simulink model "EV_Truck_Model"  (R2022b)
settings: Solver=FixedStepAuto  StartTime=0  StopTime=26553  FixedStep=0.1  RelTol=1e-3
model workspace (MAT data in the model file):
  ADAS_MaxAccel = 2
  ADAS_MaxDecel = 2.5
  Adas_on_off = 0
  Batt_cap_ah : Simulink.Parameter (value not decoded)
  Batt_rist_r0 : Simulink.Parameter (value not decoded)
  Batt_soc_s0 : Simulink.Parameter (value not decoded)
  Batt_volt_v0 : Simulink.Parameter (value not decoded)
  Motor_eff_100 : Simulink.Parameter (value not decoded)
  Motor_eff_190 : Simulink.Parameter (value not decoded)
  Motor_eff_95 : Simulink.Parameter (value not decoded)
  Motor_rpm_100 : Simulink.Parameter (value not decoded)
  Motor_rpm_190 : Simulink.Parameter (value not decoded)
  Motor_rpm_95 : Simulink.Parameter (value not decoded)
  Motor_torque_pos_100 : Simulink.Parameter (value not decoded)
  Motor_torque_pos_190 : Simulink.Parameter (value not decoded)
  Motor_torque_pos_95 : Simulink.Parameter (value not decoded)
  Motor_trq_190 : Simulink.Parameter (value not decoded)
  Motor_trq_95 : Simulink.Parameter (value not decoded)
  Sim_step = 0.1
  Test_DriveCycle = 0
  Trans_ratio = 6.142
  Veh_cog_fx = 1.69543
  Veh_cog_h = 0.605887
  Veh_cog_rx = 2.11956
  Veh_diff = 6.7
  Veh_whl_crr = 0.01
  Veh_whl_k = 180000
  Veh_whl_radius = 0.35
symbols that are objects in the model workspace (value not decoded): Motor_eff_100, Motor_eff_190, Motor_eff_95, Motor_rpm_100, Motor_rpm_190, Motor_rpm_95, Motor_torque_pos_100, Motor_torque_pos_190, Motor_torque_pos_95, Motor_trq_190, Motor_trq_95
undefined symbols (not defined in the file): Batt_soc_init, canChannel, Elec_aux_sw, Elec_rgn_sw, Power_option, speed, time, Veh_mass
libraries: batteryecm_lib x170, simulink x14, canmsglib x9, canlib x7, autolibshared x5, nesl_utility x4, fl_lib x3, drivingvehiclecontroller x3, hdlsllib x3, sim3dlib x1, sim3dautolib x1, vrlib x1
(part 10 of 11)

== system EV_Truck_Model/Accumulator System/Battery Pack/Simscape HV Battery/Battery Semi-Pack 4/Battery 7s6p5 ==
  Battery{1..7} (7 alike) : batteryecm_lib/Battery (Table-Based)  SOC_vec=Batt_soc_s0  T_dependence=simscape.enum.tablebattery.temperature_dependence.no  prm_dir=simscape.enum.tablebattery.prm_dir.noCurrentDirectionality  T_vec=[293] K  V0_mat=[2, 3, 3.2, 3.25, 3.25, 3.3, 3.3, 3.3, 3.35, 3.5] V  V0_vec=Batt_volt_v0 V  V_range=[0, inf] V  R0_mat=[15] mOhm  R0_vec=Batt_rist_r0 mOhm  R0_dis_mat=[.0117, .0085, .009; .011, .0085, .009; .0114, .0087, .0092; .0107, .0082, .0088; .0107, .0083, .0091; .0113, .0085, .0089; .0116, .0085, .0089] Ohm  R0_dis_vec=[.0085, .0085, .0087, .0082, .0083, .0085, .0085] Ohm  R0_ch_mat=[.0117, .0085, .009; .011, .0085, .009; .0114, .0087, .0092; .0107, .0082, .0088; .0107, .0083, .0091; .0113, .0085, .0089; .0116, .0085, .0089] Ohm  R0_ch_vec=[.0085, .0085, .0087, .0082, .0083, .0085, .0085] Ohm  AH=Batt_cap_ah A*hr  prm_leak=simscape.enum.tablebattery.prm_leak.disabled  Rleak_vec=[8000, 7000, 6000] Ohm  Rleak=7e3 Ohm  extrapolation_option=simscape.enum.extrapolation.nearest  SOC_port=simscape.enum.tablebattery.enable.no  prm_dyn=simscape.enum.tablebattery.prm_dyn.off  R1_mat=[.0109, .0029, .0013; .0069, .0024, .0012; .0047, .0026, .0013; .0034, .0016, .001; .0033, .0023, .0014; .0033, .0018, .0011; .0028, .0017, .0011] Ohm  R1_vec=[.0029, .0024, .0026, .0016, .0023, .0018, .0017] Ohm  tau1_mat=[20, 36, 39; 31, 45, 39; 109, 105, 61; 36, 29, 26; 59, 77, 67; 40, 33, 29; 25, 39, 33] s  tau1_vec=[36, 45, 105, 29, 77, 33, 39] s  R2_mat=[.0109, .0029, .0013; .0069, .0024, .0012; .0047, .0026, .0013; .0034, .0016, .001; .0033, .0023, .0014; .0033, .0018, .0011; .0028, .0017, .0011] Ohm  R2_vec=[.0029, .0024, .0026, .0016, .0023, .0018, .0017] Ohm  tau2_mat=[20, 36, 39; 31, 45, 39; 109, 105, 61; 36, 29, 26; 59, 77, 67; 40, 33, 29; 25, 39, 33] s  tau2_vec=[36, 45, 105, 29, 77, 33, 39] s  R3_mat=[.0109, .0029, .0013; .0069, .0024, .0012; .0047, .0026, .0013; .0034, .0016, .001; .0033, .0023, .0014; .0033, .0018, .0011; .0028, .0017, .0011] Ohm  R3_vec=[.0029, .0024, .0026, .0016, .0023, .0018, .0017] Ohm  tau3_mat=[20, 36, 39; 31, 45, 39; 109, 105, 61; 36, 29, 26; 59, 77, 67; 40, 33, 29; 25, 39, 33] s  tau3_vec=[36, 45, 105, 29, 77, 33, 39] s  R4_mat=[.0109, .0029, .0013; .0069, .0024, .0012; .0047, .0026, .0013; .0034, .0016, .001; .0033, .0023, .0014; .0033, .0018, .0011; .0028, .0017, .0011] Ohm  R4_vec=[.0029, .0024, .0026, .0016, .0023, .0018, .0017] Ohm  tau4_mat=[20, 36, 39; 31, 45, 39; 109, 105, 61; 36, 29, 26; 59, 77, 67; 40, 33, 29; 25, 39, 33] s  tau4_vec=[36, 45, 105, 29, 77, 33, 39] s  R5_mat=[.0109, .0029, .0013; .0069, .0024, .0012; .0047, .0026, .0013; .0034, .0016, .001; .0033, .0023, .0014; .0033, .0018, .0011; .0028, .0017, .0011] Ohm  R5_vec=[.0029, .0024, .0026, .0016, .0023, .0018, .0017] Ohm  tau5_mat=[20, 36, 39; 31, 45, 39; 109, 105, 61; 36, 29, 26; 59, 77, 67; 40, 33, 29; 25, 39, 33] s  tau5_vec=[36, 45, 105, 29, 77, 33, 39] s  prm_fade=simscape.enum.tablebattery.prm_fade.disabled  N0=100  dV0=0  dR0=0  dAH=0  dRleak=0  dR1=0  dR2=0  dR3=0  dR4=0  dR5=0  N0vec=[100, 200, 300]  Tfadevec=[298.15, 323.15] K  dV0vec=[0, 0, 0]  dR0vec=[0, 0, 0]  dAHvec=[0, 0, 0]  dRleakvec=[0, 0, 0]  dR1vec=[0, 0, 0]  dR2vec=[0, 0, 0]  dR3vec=[0, 0, 0]  dR4vec=[0, 0, 0]  dR5vec=[0, 0, 0]  dV0mat=[0, 0; 0, 0; 0, 0]  dR0mat=[0, 0; 0, 0; 0, 0]  dAHmat=[0, 0; 0, 0; 0, 0]  dRleakmat=[0, 0; 0, 0; 0, 0]  dR1mat=[0, 0; 0, 0; 0, 0]  dR2mat=[0, 0; 0, 0; 0, 0]  dR3mat=[0, 0; 0, 0; 0, 0]  dR4mat=[0, 0; 0, 0; 0, 0]  dR5mat=[0, 0; 0, 0; 0, 0]  prm_age_modeling=simscape.enum.tablebattery.prm_age_modeling.equation  storage_dt_age_vec=[0] d  storage_T_age_vec=[273] K  prm_age_OCV=simscape.enum.tablebattery.prm_age_OCV.OCV  OCV_age=0.9  SOC_age=0.6  prm_age_resistance=simscape.enum.tablebattery.prm_age.disabled  OCV_scaling_age_resistance=2.2134e6  OCV_offset_age_resistance=1.632e6  temp_exp_age_resistance=0.515833569 V  t_exp_age_resistance=0.75  T_age_vec_resistance=[273.15, 298.15, 323.15] K  dt_age_vec_resistance=[90, 180, 270, 360] d  dR0_age_vec=[0, 0, 0]  t_meas_dR0_age=100 d  dR0_age_mat=[0, 0, 0; 0, 0, 0; 0, 0, 0; 0, 0, 0]  prm_age_capacity=simscape.enum.tablebattery.prm_age.disabled  OCV_scaling_age_capacity=1.5097e07  OCV_offset_age_capacity=8.3625e06  temp_exp_age_capacity=0.6011 V  t_exp_age_capacity=0.75  T_age_vec_capacity=[273.15, 298.15, 323.15] K  dt_age_vec_capacity=[90, 180, 270, 360] d  dAH_age_vec=[0, 0, 0]  t_meas_dAH_age=100 d  dAH_age_mat=[0, 0, 0; 0, 0, 0; 0, 0, 0; 0, 0, 0]  thermal_port=simscape.enum.thermaleffects.omit  temperature=298.15 K  thermal_mass=100 J/K  i_specify=off  i_priority=None  i=0 A  i_nominal_specify=off  i_nominal_unit=A  i_nominal_value=1  v_specify=off  v_priority=None  v=0 V  v_nominal_specify=off  v_nominal_unit=V  v_nominal_value=1  stateOfCharge_specify=on  stateOfCharge_priority=High  stateOfCharge=Batt_soc_init  stateOfCharge_nominal_specify=off  stateOfCharge_nominal_unit=1  stateOfCharge_nominal_value=1  num_cycles_specify=off  num_cycles_priority=High  num_cycles=0  num_cycles_nominal_specify=off  num_cycles_nominal_unit=1  num_cycles_nominal_value=1  cell_temperature_specify=off  cell_temperature_priority=High  cell_temperature=298.15 K  cell_temperature_nominal_specify=off  cell_temperature_nominal_unit=K  cell_temperature_nominal_value=1
      settings: InternalSimscapePortConfiguration="{\"Bottom\":[],\"Left\":[{\"id\":\"p\",\"label\":\"+\",\"type\":\"foundation.electrical.electrical\"}],\"Right\":[{\"id\":\"n\",\"label\":\"-\",\"type\":\"foundation.electrical.electrical\"}],\"Top\":[]}"
  High : PMIOPort  Side=Left
  Low : PMIOPort  Port=2  Side=Right
  connections:
  Low/RConn1 -- Battery7/RConn1
  Battery1/LConn1 -- High/RConn1
  Battery2/LConn1 -- Battery1/RConn1
  Battery3/LConn1 -- Battery2/RConn1
  Battery4/LConn1 -- Battery3/RConn1
  Battery5/LConn1 -- Battery4/RConn1
  Battery6/LConn1 -- Battery5/RConn1
  Battery7/LConn1 -- Battery6/RConn1

== system EV_Truck_Model/Accumulator System/Battery Pack/Simscape HV Battery/Battery Semi-Pack 4/Battery 7s6p6 ==
  Battery{1..6} (6 alike) : batteryecm_lib/Battery (Table-Based)  SOC_vec=Batt_soc_s0  T_dependence=simscape.enum.tablebattery.temperature_dependence.no  prm_dir=simscape.enum.tablebattery.prm_dir.noCurrentDirectionality  T_vec=[293] K  V0_mat=[2, 3, 3.2, 3.25, 3.25, 3.3, 3.3, 3.3, 3.35, 3.5] V  V0_vec=Batt_volt_v0 V  V_range=[0, inf] V  R0_mat=[15] mOhm  R0_vec=Batt_rist_r0 mOhm  R0_dis_mat=[.0117, .0085, .009; .011, .0085, .009; .0114, .0087, .0092; .0107, .0082, .0088; .0107, .0083, .0091; .0113, .0085, .0089; .0116, .0085, .0089] Ohm  R0_dis_vec=[.0085, .0085, .0087, .0082, .0083, .0085, .0085] Ohm  R0_ch_mat=[.0117, .0085, .009; .011, .0085, .009; .0114, .0087, .0092; .0107, .0082, .0088; .0107, .0083, .0091; .0113, .0085, .0089; .0116, .0085, .0089] Ohm  R0_ch_vec=[.0085, .0085, .0087, .0082, .0083, .0085, .0085] Ohm  AH=Batt_cap_ah A*hr  prm_leak=simscape.enum.tablebattery.prm_leak.disabled  Rleak_vec=[8000, 7000, 6000] Ohm  Rleak=7e3 Ohm  extrapolation_option=simscape.enum.extrapolation.nearest  SOC_port=simscape.enum.tablebattery.enable.no  prm_dyn=simscape.enum.tablebattery.prm_dyn.off  R1_mat=[.0109, .0029, .0013; .0069, .0024, .0012; .0047, .0026, .0013; .0034, .0016, .001; .0033, .0023, .0014; .0033, .0018, .0011; .0028, .0017, .0011] Ohm  R1_vec=[.0029, .0024, .0026, .0016, .0023, .0018, .0017] Ohm  tau1_mat=[20, 36, 39; 31, 45, 39; 109, 105, 61; 36, 29, 26; 59, 77, 67; 40, 33, 29; 25, 39, 33] s  tau1_vec=[36, 45, 105, 29, 77, 33, 39] s  R2_mat=[.0109, .0029, .0013; .0069, .0024, .0012; .0047, .0026, .0013; .0034, .0016, .001; .0033, .0023, .0014; .0033, .0018, .0011; .0028, .0017, .0011] Ohm  R2_vec=[.0029, .0024, .0026, .0016, .0023, .0018, .0017] Ohm  tau2_mat=[20, 36, 39; 31, 45, 39; 109, 105, 61; 36, 29, 26; 59, 77, 67; 40, 33, 29; 25, 39, 33] s  tau2_vec=[36, 45, 105, 29, 77, 33, 39] s  R3_mat=[.0109, .0029, .0013; .0069, .0024, .0012; .0047, .0026, .0013; .0034, .0016, .001; .0033, .0023, .0014; .0033, .0018, .0011; .0028, .0017, .0011] Ohm  R3_vec=[.0029, .0024, .0026, .0016, .0023, .0018, .0017] Ohm  tau3_mat=[20, 36, 39; 31, 45, 39; 109, 105, 61; 36, 29, 26; 59, 77, 67; 40, 33, 29; 25, 39, 33] s  tau3_vec=[36, 45, 105, 29, 77, 33, 39] s  R4_mat=[.0109, .0029, .0013; .0069, .0024, .0012; .0047, .0026, .0013; .0034, .0016, .001; .0033, .0023, .0014; .0033, .0018, .0011; .0028, .0017, .0011] Ohm  R4_vec=[.0029, .0024, .0026, .0016, .0023, .0018, .0017] Ohm  tau4_mat=[20, 36, 39; 31, 45, 39; 109, 105, 61; 36, 29, 26; 59, 77, 67; 40, 33, 29; 25, 39, 33] s  tau4_vec=[36, 45, 105, 29, 77, 33, 39] s  R5_mat=[.0109, .0029, .0013; .0069, .0024, .0012; .0047, .0026, .0013; .0034, .0016, .001; .0033, .0023, .0014; .0033, .0018, .0011; .0028, .0017, .0011] Ohm  R5_vec=[.0029, .0024, .0026, .0016, .0023, .0018, .0017] Ohm  tau5_mat=[20, 36, 39; 31, 45, 39; 109, 105, 61; 36, 29, 26; 59, 77, 67; 40, 33, 29; 25, 39, 33] s  tau5_vec=[36, 45, 105, 29, 77, 33, 39] s  prm_fade=simscape.enum.tablebattery.prm_fade.disabled  N0=100  dV0=0  dR0=0  dAH=0  dRleak=0  dR1=0  dR2=0  dR3=0  dR4=0  dR5=0  N0vec=[100, 200, 300]  Tfadevec=[298.15, 323.15] K  dV0vec=[0, 0, 0]  dR0vec=[0, 0, 0]  dAHvec=[0, 0, 0]  dRleakvec=[0, 0, 0]  dR1vec=[0, 0, 0]  dR2vec=[0, 0, 0]  dR3vec=[0, 0, 0]  dR4vec=[0, 0, 0]  dR5vec=[0, 0, 0]  dV0mat=[0, 0; 0, 0; 0, 0]  dR0mat=[0, 0; 0, 0; 0, 0]  dAHmat=[0, 0; 0, 0; 0, 0]  dRleakmat=[0, 0; 0, 0; 0, 0]  dR1mat=[0, 0; 0, 0; 0, 0]  dR2mat=[0, 0; 0, 0; 0, 0]  dR3mat=[0, 0; 0, 0; 0, 0]  dR4mat=[0, 0; 0, 0; 0, 0]  dR5mat=[0, 0; 0, 0; 0, 0]  prm_age_modeling=simscape.enum.tablebattery.prm_age_modeling.equation  storage_dt_age_vec=[0] d  storage_T_age_vec=[273] K  prm_age_OCV=simscape.enum.tablebattery.prm_age_OCV.OCV  OCV_age=0.9  SOC_age=0.6  prm_age_resistance=simscape.enum.tablebattery.prm_age.disabled  OCV_scaling_age_resistance=2.2134e6  OCV_offset_age_resistance=1.632e6  temp_exp_age_resistance=0.515833569 V  t_exp_age_resistance=0.75  T_age_vec_resistance=[273.15, 298.15, 323.15] K  dt_age_vec_resistance=[90, 180, 270, 360] d  dR0_age_vec=[0, 0, 0]  t_meas_dR0_age=100 d  dR0_age_mat=[0, 0, 0; 0, 0, 0; 0, 0, 0; 0, 0, 0]  prm_age_capacity=simscape.enum.tablebattery.prm_age.disabled  OCV_scaling_age_capacity=1.5097e07  OCV_offset_age_capacity=8.3625e06  temp_exp_age_capacity=0.6011 V  t_exp_age_capacity=0.75  T_age_vec_capacity=[273.15, 298.15, 323.15] K  dt_age_vec_capacity=[90, 180, 270, 360] d  dAH_age_vec=[0, 0, 0]  t_meas_dAH_age=100 d  dAH_age_mat=[0, 0, 0; 0, 0, 0; 0, 0, 0; 0, 0, 0]  thermal_port=simscape.enum.thermaleffects.omit  temperature=298.15 K  thermal_mass=100 J/K  i_specify=off  i_priority=None  i=0 A  i_nominal_specify=off  i_nominal_unit=A  i_nominal_value=1  v_specify=off  v_priority=None  v=0 V  v_nominal_specify=off  v_nominal_unit=V  v_nominal_value=1  stateOfCharge_specify=on  stateOfCharge_priority=High  stateOfCharge=Batt_soc_init  stateOfCharge_nominal_specify=off  stateOfCharge_nominal_unit=1  stateOfCharge_nominal_value=1  num_cycles_specify=off  num_cycles_priority=High  num_cycles=0  num_cycles_nominal_specify=off  num_cycles_nominal_unit=1  num_cycles_nominal_value=1  cell_temperature_specify=off  cell_temperature_priority=High  cell_temperature=298.15 K  cell_temperature_nominal_specify=off  cell_temperature_nominal_unit=K  cell_temperature_nominal_value=1
      settings: InternalSimscapePortConfiguration="{\"Bottom\":[],\"Left\":[{\"id\":\"p\",\"label\":\"+\",\"type\":\"foundation.electrical.electrical\"}],\"Right\":[{\"id\":\"n\",\"label\":\"-\",\"type\":\"foundation.electrical.electrical\"}],\"Top\":[]}"
  Battery7 : batteryecm_lib/Battery (Table-Based)  SOC_vec=Batt_soc_s0  T_dependence=simscape.enum.tablebattery.temperature_dependence.no  prm_dir=simscape.enum.tablebattery.prm_dir.noCurrentDirectionality  T_vec=[293] K  V0_mat=[2, 3, 3.2, 3.25, 3.25, 3.3, 3.3, 3.3, 3.35, 3.5] V  V0_vec=Batt_volt_v0 V  V_range=[0, inf] V  R0_mat=[15] mOhm  R0_vec=Batt_rist_r0 mOhm  R0_dis_mat=[.0117, .0085, .009; .011, .0085, .009; .0114, .0087, .0092; .0107, .0082, .0088; .0107, .0083, .0091; .0113, .0085, .0089; .0116, .0085, .0089] Ohm  R0_dis_vec=[.0085, .0085, .0087, .0082, .0083, .0085, .0085] Ohm  R0_ch_mat=[.0117, .0085, .009; .011, .0085, .009; .0114, .0087, .0092; .0107, .0082, .0088; .0107, .0083, .0091; .0113, .0085, .0089; .0116, .0085, .0089] Ohm  R0_ch_vec=[.0085, .0085, .0087, .0082, .0083, .0085, .0085] Ohm  AH=Batt_cap_ah A*hr  prm_leak=simscape.enum.tablebattery.prm_leak.disabled  Rleak_vec=[8000, 7000, 6000] Ohm  Rleak=7e3 Ohm  extrapolation_option=simscape.enum.extrapolation.nearest  SOC_port=simscape.enum.tablebattery.enable.yes  prm_dyn=simscape.enum.tablebattery.prm_dyn.off  R1_mat=[.0109, .0029, .0013; .0069, .0024, .0012; .0047, .0026, .0013; .0034, .0016, .001; .0033, .0023, .0014; .0033, .0018, .0011; .0028, .0017, .0011] Ohm  R1_vec=[.0029, .0024, .0026, .0016, .0023, .0018, .0017] Ohm  tau1_mat=[20, 36, 39; 31, 45, 39; 109, 105, 61; 36, 29, 26; 59, 77, 67; 40, 33, 29; 25, 39, 33] s  tau1_vec=[36, 45, 105, 29, 77, 33, 39] s  R2_mat=[.0109, .0029, .0013; .0069, .0024, .0012; .0047, .0026, .0013; .0034, .0016, .001; .0033, .0023, .0014; .0033, .0018, .0011; .0028, .0017, .0011] Ohm  R2_vec=[.0029, .0024, .0026, .0016, .0023, .0018, .0017] Ohm  tau2_mat=[20, 36, 39; 31, 45, 39; 109, 105, 61; 36, 29, 26; 59, 77, 67; 40, 33, 29; 25, 39, 33] s  tau2_vec=[36, 45, 105, 29, 77, 33, 39] s  R3_mat=[.0109, .0029, .0013; .0069, .0024, .0012; .0047, .0026, .0013; .0034, .0016, .001; .0033, .0023, .0014; .0033, .0018, .0011; .0028, .0017, .0011] Ohm  R3_vec=[.0029, .0024, .0026, .0016, .0023, .0018, .0017] Ohm  tau3_mat=[20, 36, 39; 31, 45, 39; 109, 105, 61; 36, 29, 26; 59, 77, 67; 40, 33, 29; 25, 39, 33] s  tau3_vec=[36, 45, 105, 29, 77, 33, 39] s  R4_mat=[.0109, .0029, .0013; .0069, .0024, .0012; .0047, .0026, .0013; .0034, .0016, .001; .0033, .0023, .0014; .0033, .0018, .0011; .0028, .0017, .0011] Ohm  R4_vec=[.0029, .0024, .0026, .0016, .0023, .0018, .0017] Ohm  tau4_mat=[20, 36, 39; 31, 45, 39; 109, 105, 61; 36, 29, 26; 59, 77, 67; 40, 33, 29; 25, 39, 33] s  tau4_vec=[36, 45, 105, 29, 77, 33, 39] s  R5_mat=[.0109, .0029, .0013; .0069, .0024, .0012; .0047, .0026, .0013; .0034, .0016, .001; .0033, .0023, .0014; .0033, .0018, .0011; .0028, .0017, .0011] Ohm  R5_vec=[.0029, .0024, .0026, .0016, .0023, .0018, .0017] Ohm  tau5_mat=[20, 36, 39; 31, 45, 39; 109, 105, 61; 36, 29, 26; 59, 77, 67; 40, 33, 29; 25, 39, 33] s  tau5_vec=[36, 45, 105, 29, 77, 33, 39] s  prm_fade=simscape.enum.tablebattery.prm_fade.disabled  N0=100  dV0=0  dR0=0  dAH=0  dRleak=0  dR1=0  dR2=0  dR3=0  dR4=0  dR5=0  N0vec=[100, 200, 300]  Tfadevec=[298.15, 323.15] K  dV0vec=[0, 0, 0]  dR0vec=[0, 0, 0]  dAHvec=[0, 0, 0]  dRleakvec=[0, 0, 0]  dR1vec=[0, 0, 0]  dR2vec=[0, 0, 0]  dR3vec=[0, 0, 0]  dR4vec=[0, 0, 0]  dR5vec=[0, 0, 0]  dV0mat=[0, 0; 0, 0; 0, 0]  dR0mat=[0, 0; 0, 0; 0, 0]  dAHmat=[0, 0; 0, 0; 0, 0]  dRleakmat=[0, 0; 0, 0; 0, 0]  dR1mat=[0, 0; 0, 0; 0, 0]  dR2mat=[0, 0; 0, 0; 0, 0]  dR3mat=[0, 0; 0, 0; 0, 0]  dR4mat=[0, 0; 0, 0; 0, 0]  dR5mat=[0, 0; 0, 0; 0, 0]  prm_age_modeling=simscape.enum.tablebattery.prm_age_modeling.equation  storage_dt_age_vec=[0] d  storage_T_age_vec=[273] K  prm_age_OCV=simscape.enum.tablebattery.prm_age_OCV.OCV  OCV_age=0.9  SOC_age=0.6  prm_age_resistance=simscape.enum.tablebattery.prm_age.disabled  OCV_scaling_age_resistance=2.2134e6  OCV_offset_age_resistance=1.632e6  temp_exp_age_resistance=0.515833569 V  t_exp_age_resistance=0.75  T_age_vec_resistance=[273.15, 298.15, 323.15] K  dt_age_vec_resistance=[90, 180, 270, 360] d  dR0_age_vec=[0, 0, 0]  t_meas_dR0_age=100 d  dR0_age_mat=[0, 0, 0; 0, 0, 0; 0, 0, 0; 0, 0, 0]  prm_age_capacity=simscape.enum.tablebattery.prm_age.disabled  OCV_scaling_age_capacity=1.5097e07  OCV_offset_age_capacity=8.3625e06  temp_exp_age_capacity=0.6011 V  t_exp_age_capacity=0.75  T_age_vec_capacity=[273.15, 298.15, 323.15] K  dt_age_vec_capacity=[90, 180, 270, 360] d  dAH_age_vec=[0, 0, 0]  t_meas_dAH_age=100 d  dAH_age_mat=[0, 0, 0; 0, 0, 0; 0, 0, 0; 0, 0, 0]  thermal_port=simscape.enum.thermaleffects.omit  temperature=298.15 K  thermal_mass=100 J/K  i_specify=off  i_priority=None  i=0 A  i_nominal_specify=off  i_nominal_unit=A  i_nominal_value=1  v_specify=off  v_priority=None  v=0 V  v_nominal_specify=off  v_nominal_unit=V  v_nominal_value=1  stateOfCharge_specify=on  stateOfCharge_priority=High  stateOfCharge=Batt_soc_init  stateOfCharge_nominal_specify=off  stateOfCharge_nominal_unit=1  stateOfCharge_nominal_value=1  num_cycles_specify=off  num_cycles_priority=High  num_cycles=0  num_cycles_nominal_specify=off  num_cycles_nominal_unit=1  num_cycles_nominal_value=1  cell_temperature_specify=off  cell_temperature_priority=High  cell_temperature=298.15 K  cell_temperature_nominal_specify=off  cell_temperature_nominal_unit=K  cell_temperature_nominal_value=1
      settings: InternalSimscapePortConfiguration="{\"Bottom\":[],\"Left\":[{\"id\":\"p\",\"label\":\"+\",\"type\":\"foundation.electrical.electrical\"},{\"id\":\"soc\",\"label\":\"SOC\",\"type\":\"output\"}],\"Right\":[{\"id\":\"n\",\"label\":\"-\",\"type\":\"foundation.electrical.electrical\"}],\"Top\":[]}"
  High : PMIOPort  Side=Left
  Low : PMIOPort  Port=2  Side=Right
  SOC : PMIOPort  Port=3  Side=Left
  connections:
  Low/RConn1 -- Battery7/RConn1
  Battery1/LConn1 -- High/RConn1
  Battery2/LConn1 -- Battery1/RConn1
  Battery3/LConn1 -- Battery2/RConn1
  Battery4/LConn1 -- Battery3/RConn1
  Battery5/LConn1 -- Battery4/RConn1
  Battery6/LConn1 -- Battery5/RConn1
  Battery7/LConn1 -- Battery6/RConn1
  Battery7/LConn2 -- SOC/RConn1

== system EV_Truck_Model/VCU/Remap Subsystem/Longitudinal Control Subsystem/If Action Subsystem/ADAS Torque Command MUX ==
  TrqCmd : Inport
  BrakeCmd : Inport  Port=2
  TrqCmd_ADAS : Inport  Port=3
  BrakeCmd_ADAS : Inport  Port=4
  Constant : Constant  Value=0
  If : If  IfExpression=u1 == 1
  If Action Subsystem : Subsystem  TreatAsAtomicUnit=on
  If Action Subsystem1 : Subsystem  TreatAsAtomicUnit=on
  Merge : Merge
  Merge1 : Merge
  TrqCmd_MUX : Outport
  BrakeCmd_MUX : Outport  Port=2
  wires:
  TrqCmd/1 -> If Action Subsystem/1(TrqCmd)
  If Action Subsystem/1(Out1) -> Merge/1
  TrqCmd_ADAS/1 -> If Action Subsystem1/1(TrqCmd_ADAS)
  If Action Subsystem1/1(Out1) -> Merge/2
  Constant/1 -> If/1
  If/1 -> If Action Subsystem1/Action
  If/2 -> If Action Subsystem/Action
  Merge/1 -> TrqCmd_MUX/1
  BrakeCmd/1 -> If Action Subsystem/2(BrakeCmd)
  BrakeCmd_ADAS/1 -> If Action Subsystem1/2(BrakeCmd_ADAS)
  Merge1/1 -> BrakeCmd_MUX/1
  If Action Subsystem1/2(Out2) -> Merge1/2
  If Action Subsystem/2(Out2) -> Merge1/1

== system EV_Truck_Model/VCU/Remap Subsystem/Longitudinal Controller/ADAS Torque Command MUX/If Action Subsystem ==
  TrqCmd : Inport
  BrakeCmd : Inport  Port=2
  Action Port : ActionPort  ActionPortLabel=else
  Out1 : Outport
  Out2 : Outport  Port=2
  wires:
  TrqCmd/1 -> Out1/1
  BrakeCmd/1 -> Out2/1

== system EV_Truck_Model/VCU/Remap Subsystem/Longitudinal Controller/ADAS Torque Command MUX/If Action Subsystem1 ==
  TrqCmd_ADAS : Inport
  BrakeCmd_ADAS : Inport  Port=2
  Action Port : ActionPort  ActionPortLabel=if(u1 == 1)
  Out1 : Outport
  Out2 : Outport  Port=2
  wires:
  TrqCmd_ADAS/1 -> Out1/1
  BrakeCmd_ADAS/1 -> Out2/1

== system EV_Truck_Model/VCU/Remap Subsystem/TTC Calculator/Subsystem/Subsystem ==
  In1 : Inport
  In2 : Inport  Port=2
  Constant : Constant
  Delay : Delay  DelayLengthSource=Input port  DelayLength=1
      settings: InputPortMap=u0,p1
  Delay1 : Delay  DelayLengthSource=Input port  DelayLength=1
      settings: InputPortMap=u0,p1
  Divide : Product  Inputs=*/
  Minus : Sum  Inputs=+-
  Minus1 : Sum  Inputs=+-
  Out1 : Outport
  wires:
  Minus/1 -> Divide/1
  Delay/1 -> Minus/2
  In1/1 -> Minus/1, Delay/1
  Delay1/1 -> Minus1/2
  In2/1 -> Delay1/1, Minus1/1
  Minus1/1 -> Divide/2
  Divide/1 -> Out1/1
  Constant/1 -> Delay1/2, Delay/2

== system EV_Truck_Model/VCU/Remap Subsystem/TTC Calculator/Subsystem/Subsystem1 ==
  In1 : Inport
  In2 : Inport  Port=2
  Constant : Constant  Value=2
  Delay : Delay  DelayLengthSource=Input port  DelayLength=1
      settings: InputPortMap=u0,p1
  Delay1 : Delay  DelayLengthSource=Input port  DelayLength=1
      settings: InputPortMap=u0,p1
  Divide : Product  Inputs=*/
  Minus : Sum  Inputs=+-
  Minus1 : Sum  Inputs=+-
  Out1 : Outport
  wires:
  Minus/1 -> Divide/1
  Delay/1 -> Minus/2
  In1/1 -> Minus/1, Delay/1
  Delay1/1 -> Minus1/2
  In2/1 -> Delay1/1, Minus1/1
  Minus1/1 -> Divide/2
  Divide/1 -> Out1/1
  Constant/1 -> Delay1/2, Delay/2

== system EV_Truck_Model/VCU/Remap Subsystem/TTC Calculator/Subsystem/Subsystem2 ==
  In1 : Inport
  In2 : Inport  Port=2
  Constant : Constant  Value=3
  Delay : Delay  DelayLengthSource=Input port  DelayLength=1
      settings: InputPortMap=u0,p1
  Delay1 : Delay  DelayLengthSource=Input port  DelayLength=1
      settings: InputPortMap=u0,p1
  Divide : Product  Inputs=*/
  Minus : Sum  Inputs=+-
  Minus1 : Sum  Inputs=+-
  Out1 : Outport
  wires:
  Minus/1 -> Divide/1
  Delay/1 -> Minus/2
  In1/1 -> Minus/1, Delay/1
  Delay1/1 -> Minus1/2
  In2/1 -> Delay1/1, Minus1/1
  Minus1/1 -> Divide/2
  Divide/1 -> Out1/1
  Constant/1 -> Delay1/2, Delay/2

== system EV_Truck_Model/VCU/Remap Subsystem/TTC Calculator/Subsystem/Subsystem3 ==
  In1 : Inport
  In2 : Inport  Port=2
  Constant : Constant  Value=4
  Delay : Delay  DelayLengthSource=Input port  DelayLength=1
      settings: InputPortMap=u0,p1
  Delay1 : Delay  DelayLengthSource=Input port  DelayLength=1
      settings: InputPortMap=u0,p1
  Divide : Product  Inputs=*/
  Minus : Sum  Inputs=+-
  Minus1 : Sum  Inputs=+-
  Out1 : Outport
  wires:
  Minus/1 -> Divide/1
  Delay/1 -> Minus/2
  In1/1 -> Minus/1, Delay/1
  Delay1/1 -> Minus1/2
  In2/1 -> Delay1/1, Minus1/1
  Minus1/1 -> Divide/2
  Divide/1 -> Out1/1
  Constant/1 -> Delay1/2, Delay/2

== system EV_Truck_Model/VCU/Remap Subsystem/TTC Calculator/Subsystem/Subsystem4 ==
  In1 : Inport
  In2 : Inport  Port=2
  Constant : Constant  Value=5
  Delay : Delay  DelayLengthSource=Input port  DelayLength=1
      settings: InputPortMap=u0,p1
  Delay1 : Delay  DelayLengthSource=Input port  DelayLength=1
      settings: InputPortMap=u0,p1
  Divide : Product  Inputs=*/
  Minus : Sum  Inputs=+-
  Minus1 : Sum  Inputs=+-
  Out1 : Outport
  wires:
  Minus/1 -> Divide/1
  Delay/1 -> Minus/2
  In1/1 -> Minus/1, Delay/1
  Delay1/1 -> Minus1/2
  In2/1 -> Delay1/1, Minus1/1
  Minus1/1 -> Divide/2
  Divide/1 -> Out1/1
  Constant/1 -> Delay1/2, Delay/2

== system EV_Truck_Model/Vehicle Dynamics System/Power Delivery and Braking System/BrakeSystem & Tyre Rolling Resistance/Subsystem/If Action Subsystem ==
  MotorSpeed : Inport
  BrakingForce : Inport  Port=2
  Action Port : ActionPort  ActionPortLabel=if((-125 < u1) & (u1 < 125))
  Multiply : Gain  Gain=-1/125
  multiply : Product  Inputs=**
  Out1 : Outport
  wires:
  multiply/1 -> Multiply/1
  BrakingForce/1 -> multiply/2
  MotorSpeed/1 -> multiply/1
  Multiply/1 -> Out1/1

== system EV_Truck_Model/Vehicle Dynamics System/Power Delivery and Braking System/BrakeSystem & Tyre Rolling Resistance/Subsystem/If Action Subsystem1 ==
  BrakingForce : Inport
  Action Port : ActionPort  ActionPortLabel=elseif(u1 > 0)
  Multiply : Gain  Gain=-1
  Out1 : Outport
  wires:
  BrakingForce/1 -> Multiply/1
  Multiply/1 -> Out1/1

== system EV_Truck_Model/Vehicle Dynamics System/Power Delivery and Braking System/BrakeSystem & Tyre Rolling Resistance/Subsystem/If Action Subsystem2 ==
  BrakingForce : Inport
  Action Port : ActionPort  ActionPortLabel=elseif(u1 < 0)
  Multiply : Gain
  Out1 : Outport
  wires:
  BrakingForce/1 -> Multiply/1
  Multiply/1 -> Out1/1

== system EV_Truck_Model/VCU/Remap Subsystem/Longitudinal Control Subsystem/If Action Subsystem/ADAS Torque Command MUX/If Action Subsystem ==
  TrqCmd : Inport
  BrakeCmd : Inport  Port=2
  Action Port : ActionPort
  Out1 : Outport
  Out2 : Outport  Port=2
  wires:
  TrqCmd/1 -> Out1/1
  BrakeCmd/1 -> Out2/1

== system EV_Truck_Model/VCU/Remap Subsystem/Longitudinal Control Subsystem/If Action Subsystem/ADAS Torque Command MUX/If Action Subsystem1 ==
  TrqCmd_ADAS : Inport
  BrakeCmd_ADAS : Inport  Port=2
  Action Port : ActionPort
  Out1 : Outport
  Out2 : Outport  Port=2
  wires:
  TrqCmd_ADAS/1 -> Out1/1
  BrakeCmd_ADAS/1 -> Out2/1

== matlab function EV_Truck_Model/Drive Cycle and Visualization/MATLAB Function ==
  data: u input; y output
function y = fcn(u)
y = zeros(5,3);
y(1,1) = u;

== stateflow chart EV_Truck_Model/System I//O/Controller Remap/Controller Mapping ==
  state ACC
    acc = -data;
    brk = 0;
  state NC
    acc = 0;
    brk = 0;
  state BRK
    acc = 0;
    brk = data;
  note: data range: -1(Full THR)~1(Full BRK)
  (default) -> ACC
  NC -> (junction 9)
  (junction 9) -> ACC [order 3] : [data < -0.005]
  ACC -> (junction 9)
  (junction 9) -> NC [order 1] : [-0.005 <= data <= 0.005]
  BRK -> (junction 9)
  (junction 9) -> BRK [order 2] : [data > 0.005]
  data: acc output; brk output; data input
